simulink model "LRC_Phase2_OpenLoop"  (R2026a)
settings: Solver=ode45  StartTime=0  StopTime=1  MaxStep=0.001  RelTol=1e-8  AbsTol=1e-10
model workspace (MAT data in the model file):
  C = 0.00051
  E = 1.53
  L = 1
  R = 10
  Req = 40
settings Model: Creator=yogeshkhatrichhetri  LastModifiedBy=yogeshkhatrichhetri
settings DataIOCC: SaveState=on

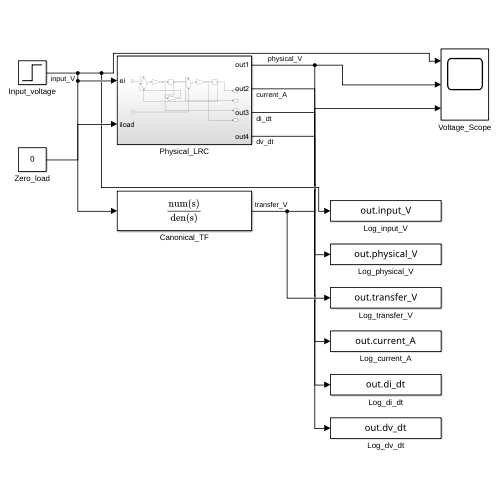
[thumbnail: Simulink's stored preview of the top-level diagram]
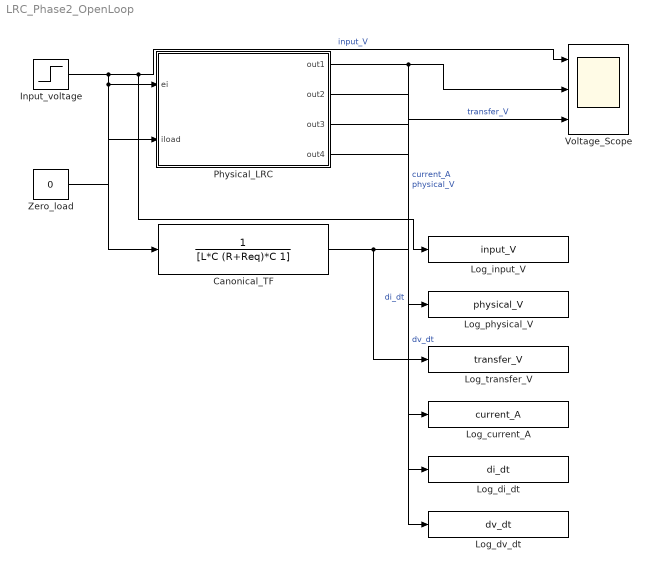
== system LRC_Phase2_OpenLoop ==
  Canonical_TF : TransferFcn  Numerator=1  Denominator=[L*C (R+Req)*C 1]
  Input_voltage : Step  Time=0  FinalValue=E  SampleTime=0
  Log_current_A : ToWorkspace  VariableName=current_A  SaveFormat=Timeseries  SampleTime=-1
  Log_di_dt : ToWorkspace  VariableName=di_dt  SaveFormat=Timeseries  SampleTime=-1
  Log_dv_dt : ToWorkspace  VariableName=dv_dt  SaveFormat=Timeseries  SampleTime=-1
  Log_input_V : ToWorkspace  VariableName=input_V  SaveFormat=Timeseries  SampleTime=-1
  Log_physical_V : ToWorkspace  VariableName=physical_V  SaveFormat=Timeseries  SampleTime=-1
  Log_transfer_V : ToWorkspace  VariableName=transfer_V  SaveFormat=Timeseries  SampleTime=-1
  Physical_LRC : Subsystem
  Voltage_Scope : Scope  NumInputPorts=3
      settings: TimeSpan=2.5  ActiveDisplayYMinimum=-0.058818963784072364  ActiveDisplayYMaximum=1.7858807848301279
  Zero_load : Constant  Value=0
  wires:
  Input_voltage/1 -> Physical_LRC/1(ei), Canonical_TF/1, Log_input_V/1, Voltage_Scope/1  "input_V"
  Zero_load/1 -> Physical_LRC/2(iload)
  Physical_LRC/1(out1) -> Log_physical_V/1, Voltage_Scope/2  "physical_V"
  Canonical_TF/1 -> Log_transfer_V/1, Voltage_Scope/3  "transfer_V"
  Physical_LRC/2(out2) -> Log_current_A/1  "current_A"
  Physical_LRC/3(out3) -> Log_di_dt/1  "di_dt"
  Physical_LRC/4(out4) -> Log_dv_dt/1  "dv_dt"

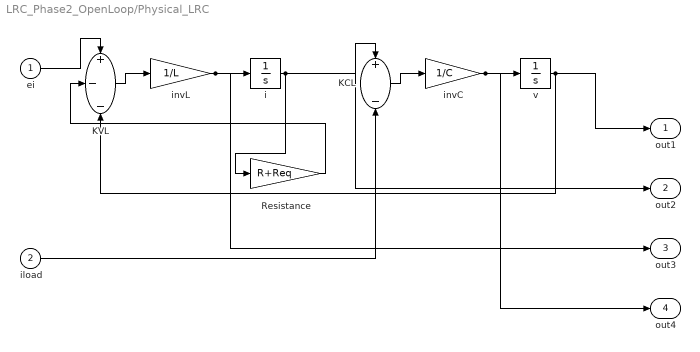
== system LRC_Phase2_OpenLoop/Physical_LRC ==
  ei : Inport
  iload : Inport  Port=2
  KCL : Sum  Inputs=+-
  KVL : Sum  Inputs=+--
  Resistance : Gain  Gain=R+Req
  i : Integrator
  invC : Gain  Gain=1/C
  invL : Gain  Gain=1/L
  v : Integrator
  out1 : Outport
  out2 : Outport  Port=2
  out3 : Outport  Port=3
  out4 : Outport  Port=4
  wires:
  ei/1 -> KVL/1
  Resistance/1 -> KVL/2
  v/1 -> KVL/3, out1/1
  KVL/1 -> invL/1
  invL/1 -> i/1, out3/1
  i/1 -> Resistance/1, KCL/1, out2/1
  iload/1 -> KCL/2
  KCL/1 -> invC/1
  invC/1 -> v/1, out4/1
